simulink model "Modelo_revision2"  (R2025b)
settings: Solver=ode3  StartTime=0  StopTime=10  FixedStep=0.001  RelTol=1e-3
model workspace (MAT data in the model file):
  A = 14.657405763
  B = 14.9893999999
  B1 = 0
  B2 = 1500
  C = 4999.99999988
  K1 = 160000
  K2 = 16000
  Kd = 7251.58073434
  Ki = 175873.08249
  Kp = 87476.5519442
  M1 = 50
  M2 = 250
  Ts = 10
libraries: simulink x2, fuzblock x1, slpidlib x1
settings Model: Creator=bug  LastModifiedBy=bug

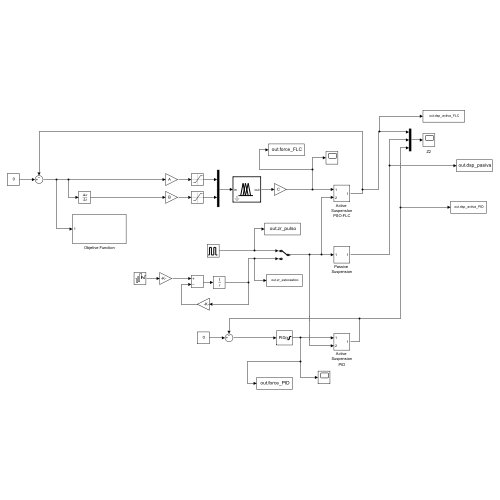
[thumbnail: Simulink's stored preview of the top-level diagram]
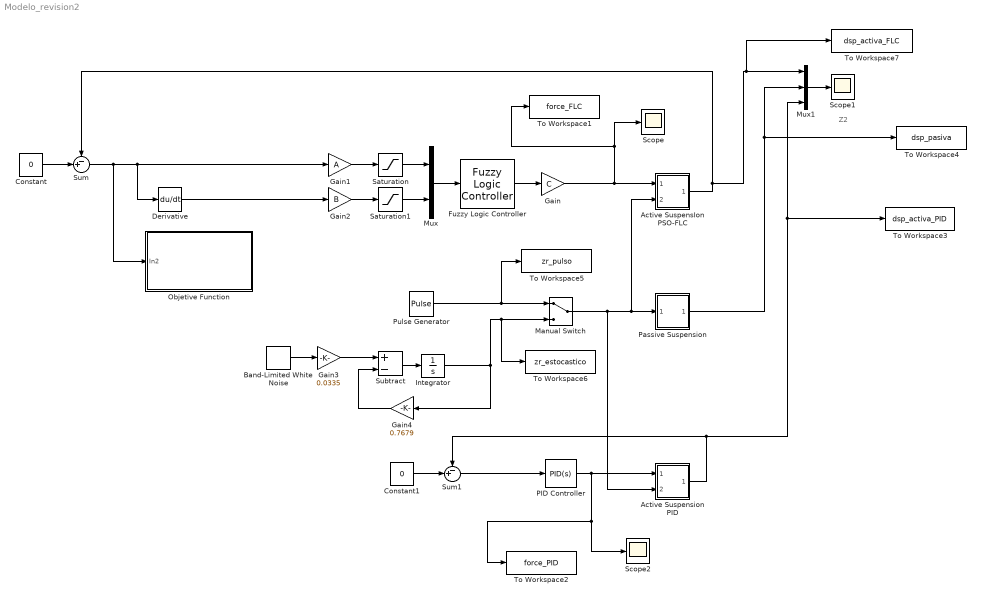
== system Modelo_revision2 ==
  note: Z2
  Active SuspensIon PSO-FLC : Subsystem
  Active Suspension PID : Subsystem
  Band-Limited White Noise : simulink/Sources/Band-Limited White Noise  Cov=[1]  Ts=0.001  seed=[23341]
  Constant : Constant  Value=0
  Constant1 : Constant  Value=0
  Derivative : Derivative
  Fuzzy Logic Controller : fuzblock/Fuzzy Logic  Controller  FIS='suspension.fis'  OutputSampleNumber=101  DataType=double  UseLookupTable=off  NumBreakpoints=10  FuzzifiedInputs=off  RuleFiringStrengths=off  RuleOutputs=off  AggregatedOutputs=off  SimulateUsing=Interpreted execution  OutOfRangeInputValueMessage=warning  NoRuleFiredMessage=warning  EmptyOutputFuzzySetMessage=warning
  Gain : Gain  Gain=C
  Gain1 : Gain  Gain=A
  Gain2 : Gain  Gain=B
  Gain3 : Gain  Gain=0.0335
  Gain4 : Gain  Gain=0.7679
  Integrator : Integrator
  Manual Switch : ManualSwitch
  Mux : Mux  Inputs=2
  Mux1 : Mux  Inputs=3
  Objetive Function : Subsystem
  PID Controller : slpidlib/PID Controller  Controller=PID  Form=Parallel  TimeDomain=Continuous-time  UseExternalTs=off  SampleTime=-1  IntegratorMethod=Forward Euler  FilterMethod=Forward Euler  ControllerParametersSource=internal  P=Kp  I=Ki  UseKiTs=off  D=Kd  UseExternalDerivativeSource=off  N=200  UseFilter=on  TunerSelectOption=Transfer Function Based (PID Tuner App)  InitialConditionSource=internal  InitialConditionForIntegrator=0  InitialConditionForFilter=0  DifferentiatorICPrevScaledInput=0  ExternalReset=none  TrackingMode=off  Kt=1  LimitOutput=on  SatLimitsSource=internal  UpperSaturationLimit=5000  LowerSaturationLimit=-5000  LinearizeAsGain=on  AntiWindupMode=clamping  Kb=1  LimitIntegrator=off  UpperIntegratorSaturationLimit=inf  LowerIntegratorSaturationLimit=-inf  POutMin=[]  POutMax=[]  IOutMin=[]  IOutMax=[]  DOutMin=[]  DOutMax=[]  NOutMin=[]  NOutMax=[]  SumOutMin=[]  SumOutMax=[]  SaturationOutMin=[]  SaturationOutMax=[]  PParamMin=[]  PParamMax=[]  IParamMin=[]  IParamMax=[]  DParamMin=[]  DParamMax=[]  NParamMin=[]  NParamMax=[]  KbParamMin=[]  KbParamMax=[]  KtParamMin=[]  KtParamMax=[]  KbOutMin=[]  KbOutMax=[]  KtOutMin=[]  KtOutMax=[]  IntegratorOutMin=[]  IntegratorOutMax=[]  FilterOutMin=[]  FilterOutMax=[]  SumI1OutMin=[]  SumI1OutMax=[]  SumI2OutMin=[]  SumI2OutMax=[]  SumI3OutMin=[]  SumI3OutMax=[]  SumI4OutMin=[]  SumI4OutMax=[]  SumDOutMin=[]  SumDOutMax=[]  DifferentiatorOutMin=[]  DifferentiatorOutMax=[]  FilterDiffOutCoefMin=[]  FilterDiffOutCoefMax=[]  ReciprocalOutMin=[]  ReciprocalOutMax=[]  SumDenOutMin=[]  SumDenOutMax=[]  SumNumOutMin=[]  SumNumOutMax=[]  DivideOutMin=[]  DivideOutMax=[]  UdiffTsProdOutMin=[]  UdiffTsProdOutMax=[]  NTsProdOutMin=[]  NTsProdOutMax=[]  UintegralTsProdOutMin=[]  UintegralTsProdOutMax=[]  UngainTsProdOutMin=[]  UngainTsProdOutMax=[]  ClampingZeroOutDataTypeStr=Inherit: Inherit via back propagation  ClampingZeroOutMin=[]  ClampingZeroOutMax=[]  FilterDenConstantOutDataTypeStr=Inherit: Inherit via back propagation  FilterDenConstantOutMin=[]  FilterDenConstantOutMax=[]  PCopyOutDataTypeStr=Inherit: Inherit via back propagation  PCopyOutMin=[]  PCopyOutMax=[]  NCopyOutDataTypeStr=Inherit: Inherit via back propagation  NCopyOutMin=[]  NCopyOutMax=[]  IntegratorContinuousStateAttributes=''  IntegratorStateMustResolveToSignalObject=off  IntegratorRTWStateStorageClass=Auto  FilterContinuousStateAttributes=''  FilterStateMustResolveToSignalObject=off  FilterRTWStateStorageClass=Auto  ParallelPVariant=InternalParameters  IdealPVariant=Disabled  IVariant=InternalParameters  DVariant=InternalParameters  IntegratorVariant=Continuous  SatVariant=Enabled  AWVariant=ContClampingParallel  PCopyVariant=Disabled  TRVariant=Disabled  FdbkBlocksVariant=Forward  IdealPFdbkVariant=Disabled  SatFdbkVariant=Disabled  DerivativeFilterVariant=ContFilter  NVariant=InternalParameters  NCopyVariant=Disabled  FilterICVariant=InternalICsFilter  IntegratorICVariant=InternalICs  ExternalResetVariant=Disabled  TRSumVariant=Passthrough  SumFdbkVariant=Disabled  SumVariant=Sum_PID  TsampFilterVariant=InternalTs  TsampNgainVariant=Passthrough  TsampIntegralVariant=Disabled_SignalSpec  ExternalSaturationOutDataTypeStr=Inherit: Same as second input  DerivativeSourceVariant=ErrorSignal  PreIntVariant=InternalPreInt
  Passive Suspension : Subsystem
  Pulse Generator : DiscretePulseGenerator  PulseType=Time based  Amplitude=0.2  Period=10  PulseWidth=2.5  PhaseDelay=1
  Saturation : Saturate  UpperLimit=1  LowerLimit=-1
  Saturation1 : Saturate  UpperLimit=1  LowerLimit=-1
  Scope : Scope
      settings: ActiveDisplayYMinimum=-5738.6500140225917  ActiveDisplayYMaximum=5255.7141215809015
  Scope1 : Scope
      settings: ActiveDisplayYMinimum=-0.086718681634349593  ActiveDisplayYMaximum=0.089522305681078523
  Scope2 : Scope
      settings: ActiveDisplayYMinimum=-3791.4152949138743  ActiveDisplayYMaximum=1392.5036601798836  DataLoggingVariableName=ScopeData2
  Subtract : Sum  Inputs=+-
  Sum : Sum  Inputs=-+|
  Sum1 : Sum  Inputs=-+|
  To Workspace1 : ToWorkspace  VariableName=force_FLC  SaveFormat=Timeseries  SampleTime=-1
  To Workspace2 : ToWorkspace  VariableName=force_PID  SaveFormat=Timeseries  SampleTime=-1
  To Workspace3 : ToWorkspace  VariableName=dsp_activa_PID  SaveFormat=Timeseries  SampleTime=-1
  To Workspace4 : ToWorkspace  VariableName=dsp_pasiva  SaveFormat=Timeseries  SampleTime=-1
  To Workspace5 : ToWorkspace  VariableName=zr_pulso  SaveFormat=Timeseries  SampleTime=-1
  To Workspace6 : ToWorkspace  VariableName=zr_estocastico  SaveFormat=Timeseries  SampleTime=-1
  To Workspace7 : ToWorkspace  VariableName=dsp_activa_FLC  SaveFormat=Timeseries  SampleTime=-1
  wires:
  Fuzzy Logic Controller/1 -> Gain/1
  Mux/1 -> Fuzzy Logic Controller/1
  Saturation/1 -> Mux/1
  Saturation1/1 -> Mux/2
  Gain1/1 -> Saturation/1
  Gain2/1 -> Saturation1/1
  Active SuspensIon PSO-FLC/1(Out1) -> Sum/1, To Workspace7/1, Mux1/1
  Sum/1 -> Objetive Function/1(In2), Derivative/1, Gain1/1
  Constant/1 -> Sum/2
  Derivative/1 -> Gain2/1
  Mux1/1 -> Scope1/1
  Pulse Generator/1 -> To Workspace5/1, Manual Switch/1
  Manual Switch/1 -> Active SuspensIon PSO-FLC/2(In2), Passive Suspension/1(In2), Active Suspension PID/2(In2)
  Subtract/1 -> Integrator/1
  Band-Limited White Noise/1 -> Gain3/1
  Gain3/1 -> Subtract/1
  Integrator/1 -> Gain4/1, Manual Switch/2, To Workspace6/1
  Gain4/1 -> Subtract/2
  Constant1/1 -> Sum1/2
  Sum1/1 -> PID Controller/1
  PID Controller/1 -> To Workspace2/1, Scope2/1, Active Suspension PID/1(In1)
  Active Suspension PID/1(Out1) -> To Workspace3/1, Mux1/3, Sum1/1
  Gain/1 -> To Workspace1/1, Scope/1, Active SuspensIon PSO-FLC/1(In1)
  Passive Suspension/1(Out1) -> Mux1/2, To Workspace4/1

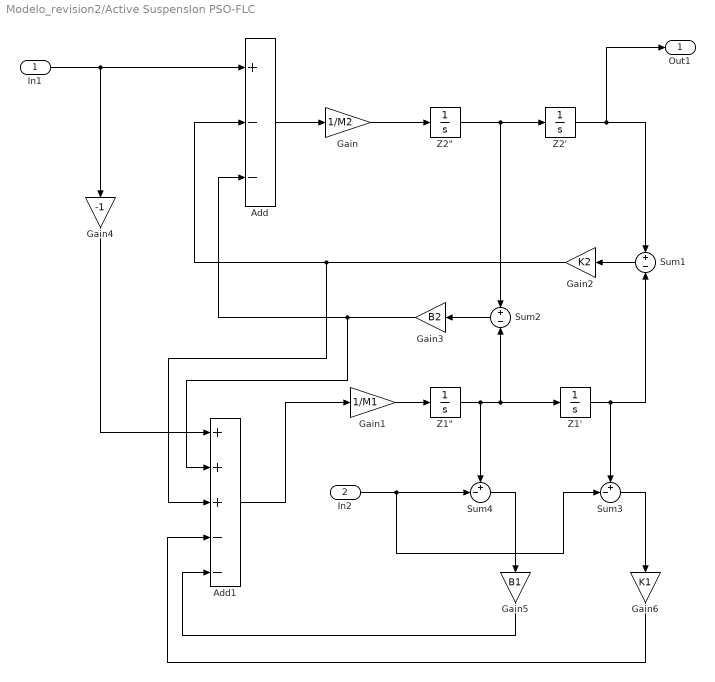
== system Modelo_revision2/Active SuspensIon PSO-FLC ==
  In1 : Inport
  In2 : Inport  Port=2
  Add : Sum  Inputs=+--
  Add1 : Sum  Inputs=+++--
  Gain : Gain  Gain=1/M2
  Gain1 : Gain  Gain=1/M1
  Gain2 : Gain  Gain=K2
  Gain3 : Gain  Gain=B2
  Gain4 : Gain  Gain=-1
  Gain5 : Gain  Gain=B1
  Gain6 : Gain  Gain=K1
  Sum1 : Sum  Inputs=+-
  Sum2 : Sum  Inputs=+-
  Sum3 : Sum  Inputs=+-|
  Sum4 : Sum  Inputs=+-|
  "Z1\"" : Integrator
  Z1' : Integrator
  "Z2\"" : Integrator
  Z2' : Integrator
  Out1 : Outport
  wires:
  Gain3/1 -> Add1/2, Add/3
  Gain2/1 -> Add/2, Add1/3
  "Z2\""/1 -> Sum2/1, Z2'/1
  Sum3/1 -> Gain6/1
  In1/1 -> Add/1, Gain4/1
  Gain1/1 -> "Z1\""/1
  "Z1\""/1 -> Sum4/1, Sum2/2, Z1'/1
  Add/1 -> Gain/1
  Add1/1 -> Gain1/1
  Sum2/1 -> Gain3/1
  Z2'/1 -> Sum1/1, Out1/1
  Sum4/1 -> Gain5/1
  Z1'/1 -> Sum3/1, Sum1/2
  In2/1 -> Sum4/2, Sum3/2
  Gain4/1 -> Add1/1
  Sum1/1 -> Gain2/1
  Gain5/1 -> Add1/5
  Gain6/1 -> Add1/4
  Gain/1 -> "Z2\""/1

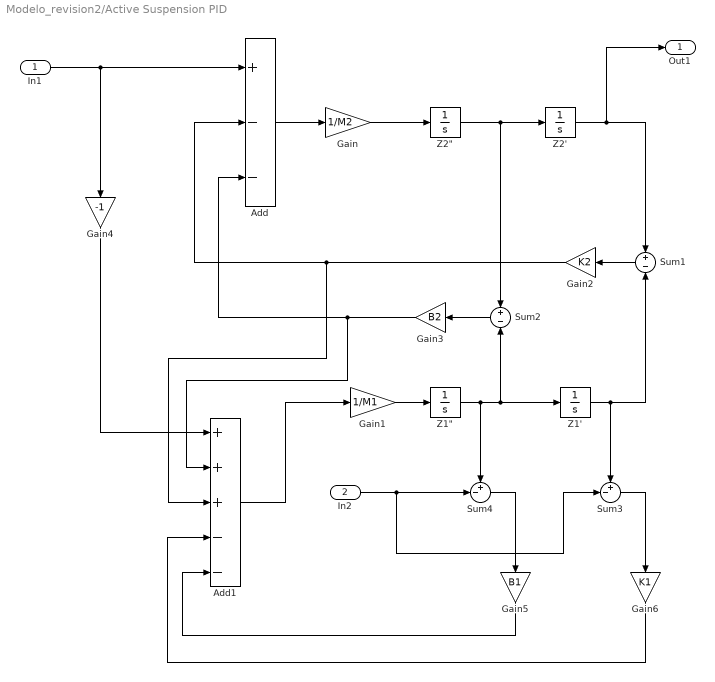
== system Modelo_revision2/Active Suspension PID ==
  In1 : Inport
  In2 : Inport  Port=2
  Add : Sum  Inputs=+--
  Add1 : Sum  Inputs=+++--
  Gain : Gain  Gain=1/M2
  Gain1 : Gain  Gain=1/M1
  Gain2 : Gain  Gain=K2
  Gain3 : Gain  Gain=B2
  Gain4 : Gain  Gain=-1
  Gain5 : Gain  Gain=B1
  Gain6 : Gain  Gain=K1
  Sum1 : Sum  Inputs=+-
  Sum2 : Sum  Inputs=+-
  Sum3 : Sum  Inputs=+-|
  Sum4 : Sum  Inputs=+-|
  "Z1\"" : Integrator
  Z1' : Integrator
  "Z2\"" : Integrator
  Z2' : Integrator
  Out1 : Outport
  wires:
  Gain3/1 -> Add1/2, Add/3
  Gain2/1 -> Add/2, Add1/3
  "Z2\""/1 -> Sum2/1, Z2'/1
  Sum3/1 -> Gain6/1
  In1/1 -> Add/1, Gain4/1
  Gain1/1 -> "Z1\""/1
  "Z1\""/1 -> Sum4/1, Sum2/2, Z1'/1
  Add/1 -> Gain/1
  Add1/1 -> Gain1/1
  Sum2/1 -> Gain3/1
  Z2'/1 -> Sum1/1, Out1/1
  Sum4/1 -> Gain5/1
  Z1'/1 -> Sum3/1, Sum1/2
  In2/1 -> Sum4/2, Sum3/2
  Gain4/1 -> Add1/1
  Sum1/1 -> Gain2/1
  Gain5/1 -> Add1/5
  Gain6/1 -> Add1/4
  Gain/1 -> "Z2\""/1

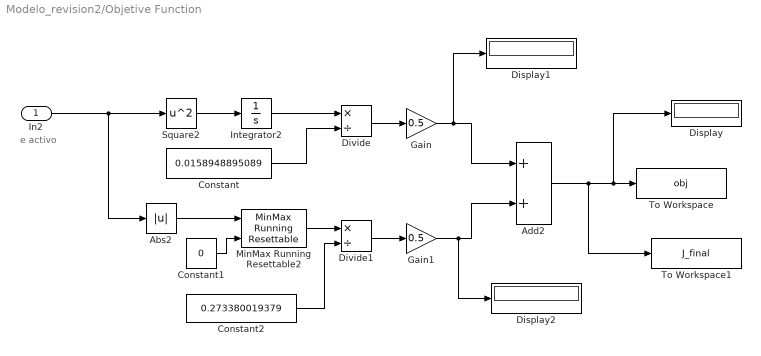
== system Modelo_revision2/Objetive Function ==
  note: e activo
  In2 : Inport
  Abs2 : Abs  SaturateOnIntegerOverflow=off
  Add2 : Sum
  Constant : Constant  Value=0.0158948895089
  Constant1 : Constant  Value=0
  Constant2 : Constant  Value=0.273380019379
  Display : Display
  Display1 : Display
  Display2 : Display
  Divide : Product  Inputs=*/
  Divide1 : Product  Inputs=*/
  Gain : Gain  Gain=0.5
  Gain1 : Gain  Gain=0.5
  Integrator2 : Integrator
  MinMax Running Resettable2 : simulink/Math Operations/MinMax Running Resettable  Function=max  vinit=0.0
  Square2 : Math  Operator=square
  To Workspace : ToWorkspace  VariableName=obj  SaveFormat=Timeseries  SampleTime=-1
  To Workspace1 : ToWorkspace  VariableName=J_final  SaveFormat=Timeseries  SampleTime=-1
  wires:
  Add2/1 -> To Workspace1/1, Display/1, To Workspace/1
  Square2/1 -> Integrator2/1
  Abs2/1 -> MinMax Running Resettable2/1
  In2/1 -> Abs2/1, Square2/1
  Constant1/1 -> MinMax Running Resettable2/2
  Integrator2/1 -> Divide/1
  MinMax Running Resettable2/1 -> Divide1/1
  Constant/1 -> Divide/2
  Constant2/1 -> Divide1/2
  Divide/1 -> Gain/1
  Divide1/1 -> Gain1/1
  Gain/1 -> Add2/1, Display1/1
  Gain1/1 -> Add2/2, Display2/1

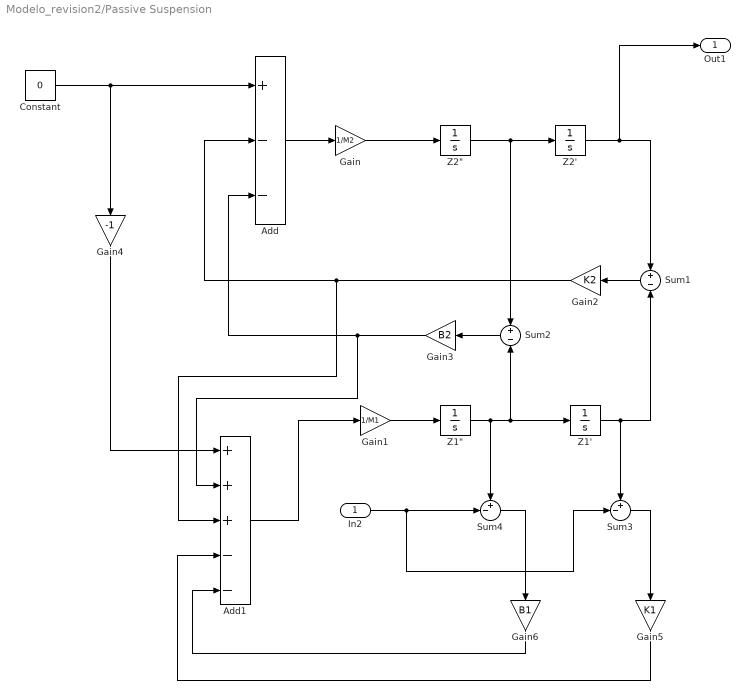
== system Modelo_revision2/Passive Suspension ==
  In2 : Inport
  Add : Sum  Inputs=+--
  Add1 : Sum  Inputs=+++--
  Constant : Constant  Value=0
  Gain : Gain  Gain=1/M2
  Gain1 : Gain  Gain=1/M1
  Gain2 : Gain  Gain=K2
  Gain3 : Gain  Gain=B2
  Gain4 : Gain  Gain=-1
  Gain5 : Gain  Gain=K1
  Gain6 : Gain  Gain=B1
  Sum1 : Sum  Inputs=+-
  Sum2 : Sum  Inputs=+-
  Sum3 : Sum  Inputs=+-|
  Sum4 : Sum  Inputs=+-|
  "Z1\"" : Integrator
  Z1' : Integrator
  "Z2\"" : Integrator
  Z2' : Integrator
  Out1 : Outport
  wires:
  Gain3/1 -> Add1/2, Add/3
  Gain2/1 -> Add/2, Add1/3
  "Z2\""/1 -> Sum2/1, Z2'/1
  Sum3/1 -> Gain5/1
  Constant/1 -> Add/1, Gain4/1
  Gain1/1 -> "Z1\""/1
  "Z1\""/1 -> Sum4/1, Sum2/2, Z1'/1
  Add/1 -> Gain/1
  Add1/1 -> Gain1/1
  Sum2/1 -> Gain3/1
  Sum4/1 -> Gain6/1
  Z1'/1 -> Sum3/1, Sum1/2
  In2/1 -> Sum4/2, Sum3/2
  Gain4/1 -> Add1/1
  Sum1/1 -> Gain2/1
  Gain5/1 -> Add1/4
  Gain6/1 -> Add1/5
  Gain/1 -> "Z2\""/1
  Z2'/1 -> Sum1/1, Out1/1
